simulink model "InductionHeating_bb_4"  (R2026b)
settings: Solver=FixedStepDiscrete  StopTime=0.008
PostLoadFcn:
  | Ts = 1e-6;Ts_fpga=10e-9;   R=3; Capa=300e-9;L=100e-6;Pejo_factor=1;
InitFcn:
  | Ts = 1e-6;Ts_fpga=10e-9;   R=3; Capa=300e-9;L=100e-6;Pejo_factor=1;
undefined symbols (not defined in the file or in its folder): DiscIntNeverNeededParam, ee_sli_rtmsupport, gcbh, isSetWhenUndefinedState, MATESOCwDio
libraries: fl_lib x67, nesl_utility x40, hdlsllib x32, simulink x15, eeGeneralControl x9, ee_lib x3
(part 2 of 7)

== system InductionHeating_bb_4/MATEwDiode ==
  note: mate_diode2.slx for diodes
  g : Inport
  Input : Inport  Port=2
  rl : Inport  Port=3
  C1 : Subsystem  AncestorBlock=simetranss/FPGA/Variable discrete RLC  mask(Discrete variable High Accuracy Series RL or Parallel RC branch){typ=Parallel RC, discmeth=Trapezoidal, Lon=1e-6, R=inf, L=10e-6, Capa=300e-9, sbrl=on, Ts=Ts, showV=off, showI=off}
      mask prompts: typ "Element type"; discmeth "Discretization"; Lon "Switch equivalent ON inductance (H)"; R "Resistor resistance (Ohms)"; L "Inductor inductance (H)"; Capa "Capacitor capacitance (F)"; sbrl "Use signal-based RLC values"; Ts "Sample Time (s)"; showV "Show voltage port"; showI "Show current port"
      mask help:
      | This model implements a discretized  Series RL or Parallel RC branch that is on-line modifiable.
      |
      | On-line modifiable:  RLC parameters can be modified during simulation.
      |
      | Choice of discretization method: Backward Euler (order 1) , Trapzoidal method (order 2) or Radau IIA (5th order)
      |
      | Use with R=0 (Series RL) to obtain a simple inductor.
      | Use with R=inf (Parallel RC) to obtain a simple capacitor.
      |
      | The block can also inplement a Pejovic Switch with the inductance parameter value for ON state. In this case, the resistance is set to 0 internally and capacitance C=Ts*Ts/L and Backward Euler is used.
      mask init:
      | block=gcb;
      | Xcomp=0;
      | s1=0;s2=0;s3=0;s4=0;r1=0;r2=0;l1=0;l2=0;
      | c1=0;c2=0;c3=0;c4=0;x1=0;x2=0;x3=0;x4=0;
      | 
      | MaskEnables =get_param (block ,'MaskEnables' ); 
      | discm=get_param(block,"discmeth");
      | if isequal(get_param(block,"discmeth"),'Backward Euler')
      |     dd=1;
      |     ddi=1;
      | elseif isequal(get_param(block,"discmeth"),'Trapezoidal')
      |     dd=2;
      |     ddi=2;
      | else
      |     dd=5;
      |     ddi=3;
      | end
      | sst=0;
      | br_typ=0;
      | is_sw=0;
      | 
      | % if isequal(get_param(block,"traprule"),'on')
      | %     Trapfactor=2;
      | % else
      | %     Trapfactor=1;
      | % end
      | RootMatch=0;
      | Ihist=0;
      | 
      | if isequal(get_param(block,"showV"),'on')
      |         replace_block (block ,'Followlinks' ,'on' ,'Name' ,'v' ,'BlockType' ,'Terminator' ,'Outport' ,'noprompt' ); 
      | else
      |         replace_block (block ,'Followlinks' ,'on' ,'Name' ,'v' ,'BlockType' ,'Outport' ,'Terminator' ,'noprompt' ); 
      | end
      | if isequal(get_param(block,"showI"),'on')
      |         replace_block (block ,'Followlinks' ,'on' ,'Name' ,'i' ,'BlockType' ,'Terminator' ,'Outport' ,'noprompt' ); 
      | else
      |         replace_block (block ,'Followlinks' ,'on' ,'Name' ,'i' ,'BlockType' ,'Outport' ,'Terminator' ,'noprompt' ); 
      | end
      | 
      | if isequal(get_param(block,"sbrl"),'on')
      |     replace_block (block ,'Followlinks' ,'on' ,'Name' ,'rlc' ,'BlockType' ,'Constant' ,'Inport' ,'noprompt' );
      |     MaskEnables {4 }='off' ;
      |     MaskEnables {5 }='off' ;
      |     MaskEnables {6 }='off' ;
      | else
      |     replace_block (block ,'Followlinks' ,'on' ,'Name' ,'rlc' ,'BlockType' ,'Inport' ,'Constant' ,'noprompt' );
      |     MaskEnables {4 }='on' ;
      |     MaskEnables {5 }='on' ;
      |     MaskEnables {6 }='on' ;
      | end
      | 
      | 
      | 
      | 
      | 
      | 
      | set_param (block ,'MaskEnables' ,MaskEnables ); 
      | qq='x';
      | 
      | typp=get_param(block,'typ');
      | % bp=get_param(block,'pcbp');
      | if isequal(typp,'Pejovic Switch')
      |     replace_block (block ,'Followlinks' ,'on' ,'Name' ,'gate' ,'BlockType' ,'Constant' ,'Inport' ,'noprompt' ); 
      |     %replace_block (block ,'Followlinks' ,'on' ,'Name' ,'init_in' ,'BlockType' ,'Inport' ,'Constant' ,'noprompt'  );
      |     %replace_block (block ,'Followlinks' ,'on' ,'Name' ,'init_out' ,'BlockType' ,'Outport' ,'Terminator' ,'noprompt'  );
      |     Rsw=Lon/Ts;
      |     txt='Switch';
      |     [s1,s2,s3,s4,r1,r2,l1,l2,c1,c2,c3,c4] = MATEdrawRLC('Series RLC Branch',0,1,0,'Open circuit');
      |     c2=[0 -20];
      |     c1=[30 120];
      |     qq='Switch';
      | % MaskEnables {2 }='on' ; 
      | % MaskEnables {3 }='off' ; 
      | % MaskEnables {4 }='off' ; 
      | % MaskEnables {5 }='off' ; 
      | % MaskEnables {6 }='off' ; 
      | % MaskEnables {8 }='off' ;
      | %force Backward Euler
      |     set_param(block,"discmeth",'Backward Euler')
      |     dd=1;
      |     ddi=1;
      |     is_sw=1;
      |     br_typ=0; % use Z=L/h 
      |  
      | elseif isequal(typp,'Inductor')
      |     replace_block (block ,'Followlinks' ,'on' ,'Name' ,'gate' ,'BlockType' ,'Inport' ,'Constant' ,'noprompt' ); 
      |     set_param([block '/gate'],'Value','1');
      |     replace_block (block ,'Followlinks' ,'on' ,'Name' ,'init_in' ,'BlockType' ,'Inport' ,'Constant' ,'noprompt'  ); 
      |     replace_block (block ,'Followlinks' ,'on' ,'Name' ,'init_out' ,'BlockType' ,'Outport' ,'Terminator' ,'noprompt'  );
      |  
      | 
      |     qq='Inductor';
      | % MaskEnables {2 }='off' ; 
      | % MaskEnables {3 }='on' ; 
      | % MaskEnables {4 }='off' ; 
      | % MaskEnables {5 }='on' ; 
      | % MaskEnables {6 }='off' ; 
      | % MaskEnables {8 }='off' ;
      |     x1=0;x2=0;x3=0;x4=0;
      |     if dd==5
      |         warning('Setting Inductor to Trapezoidal discretization');
      |         set_param(block,"discmeth",'Trapezoidal')
      |         dd=2;
      |     end
      |     [s1,s2,s3,s4,r1,r2,l1,l2,c1,c2,c3,c4] = MATEdrawRLC('Series RLC Branch',0,1,0,'L');
      |     [Ad,Bd1,Bd2,Cd,Dd,Y]=discRL(0,1/L,1,0,Ts,dd);
      |     Rsw=1/Y;
      | elseif isequal(typp,'Series RL')
      |     replace_block (block ,'Followlinks' ,'on' ,'Name' ,'gate' ,'BlockType' ,'Inport' ,'Constant' ,'noprompt' ); 
      |     set_param([block '/gate'],'Value','1');
      |     %replace_block (block ,'Followlinks' ,'on' ,'Name' ,'init_in' ,'BlockType' ,'Inport' ,'Constant' ,'noprompt'  ); 
      |     %replace_block (block ,'Followlinks' ,'on' ,'Name' ,'init_out' ,'BlockType' ,'Outport' ,'Terminator' ,'noprompt'  );
      | 
      |     [Ad,Bd1,Bd2,Cd,Dd,Y]=discRL(-R/L,1/L,1,0,Ts,dd);
      |     Rsw=1/Y;
      |     qq='Series RL';
      |     br_typ=0;
      |     sst=0;
      | % MaskEnables {2 }='off' ; 
      | % MaskEnables {3 }='on' ; 
      | % MaskEnables {4 }='off' ; 
      | if isequal(get_param(block,"sbrl"),'off')
      |   MaskEnables {4 }='on' ; 
      |   MaskEnables {5 }='on' ; 
      |   MaskEnables {6 }='off' ; 
      | end
      | % MaskEnables {8 }='off' ;
      |     x1=0;x2=0;x3=0;x4=0;
      |     [s1,s2,s3,s4,r1,r2,l1,l2,c1,c2,c3,c4] = MATEdrawRLC('Series RLC Branch',1,1,0,'RL');
      |     
      |     
      | elseif isequal(typp,'Parallel RC')
      |     replace_block (block ,'Followlinks' ,'on' ,'Name' ,'gate' ,'BlockType' ,'Inport' ,'Constant' ,'noprompt' ); 
      |     set_param([block '/gate'],'Value','0');
      |     %replace_block (block ,'Followlinks' ,'on' ,'Name' ,'init_in' ,'BlockType' ,'Inport' ,'Constant' ,'noprompt'  );
      |     %replace_block (block ,'Followlinks' ,'on' ,'Name' ,'init_out' ,'BlockType' ,'Outport' ,'Terminator' ,'noprompt'  );
      | if R<1e-6
      |     warndlg(['Resistance of RC block: ' block ' is very low for a Parallel RC Branch. Set R=inf if you really want an ideal capacitor with no parallel resistor.'],'MATE warning');
      | end
      |     qq='Capacitor';
      | % MaskEnables {2 }='off' ; 
      | % MaskEnables {3 }='off' ; 
      | % MaskEnables {4 }='on' ; 
      | if isequal(get_param(block,"sbrl"),'off')
      |   MaskEnables {4 }='on' ; 
      |   MaskEnables {5 }='off' ; 
      |   MaskEnables {6 }='on' ; 
      | end
      | 
      | % MaskEnables {8 }='off' ;
      |     % if dd==5 
      |     %     warning('Very low resistance. Setting Capacitor to Trapezoidal discretization');
      |     %     set_param(block,"discmeth",'Trapezoidal')
      |     %     dd=2;
      |     % end
      |     sst=1;
      |     br_typ=1;
      | 
      |     [Ad,Bd1,Bd2,Cd,Dd,Y]=discRL(-1/R/Capa,1/Capa,1,0,Ts,dd);
      |     Rsw=Y;
      | 
      |     if R>1e8
      |             [s1,s2,s3,s4,r1,r2,l1,l2,c1,c2,c3,c4,x1,x2,x3,x4] = MATEdrawRLC('Parallel RLC Branch',0,0,1,'C');
      |                 
      |     else
      |             [s1,s2,s3,s4,r1,r2,l1,l2,c1,c2,c3,c4,x1,x2,x3,x4] = MATEdrawRLC('Parallel RLC Branch',1,0,1,'RC');
      |                  s1=-20;s2=-120;s3=220;s4=120; %reframe
      | 
      |     end
      | 
      | 
      | elseif isequal(typp,'2-level inverter switch')
      |     replace_block (block ,'Followlinks' ,'on' ,'Name' ,'gate' ,'BlockType' ,'Constant' ,'Inport' ,'noprompt' ); 
      |     replace_block (block ,'Followlinks' ,'on' ,'Name' ,'init_in' ,'BlockType' ,'Constant' ,'Inport','noprompt'  );
      |     replace_block (block ,'Followlinks' ,'on' ,'Name' ,'init_out' ,'BlockType' ,'Terminator' ,'Outport' ,'noprompt'  );
      |     Rsw=Lon/Ts;
      |     txt='Inverter half';
      |     Xcomp=1;
      |     qq='Pejo Inverter Half';
      |     %force Backward Euler
      | set_param(block,'traprule','off');
      | % MaskEnables {2 }='on' ; 
      | % MaskEnables {3 }='off' ; 
      | % MaskEnables {4 }='off' ; 
      | % MaskEnables {5 }='off' ; 
      | % MaskEnables {6 }='off' ; 
      | % MaskEnables {8 }='on' ;
      |         [s1,s2,s3,s4,r1,r2,l1,l2,c1,c2,c3,c4] = MATEdrawRLC('Series RLC Branch',0,1,0,'Open circuit');
      |     c2=[0 -20];
      |     c1=[30 120];
      |         if dd==5  ||  dd==2
      |         set_param(block,"discmeth",'Backward Euler')
      |         dd=1;
      |         end
      | 
      | else
      | end
      | 
      | % if isequal(typp,'2-level inverter switch')  && isequal(bp,'on')
      | %         replace_block (block ,'Followlinks' ,'on' ,'Name' ,'Bypass' ,'BlockType' ,'Ground' ,'Inport' ,'noprompt' ); 
      | % else
      | %         replace_block (block ,'Followlinks' ,'on' ,'Name' ,'Bypass' ,'BlockType' ,'Inport' ,'Ground' ,'noprompt' ); 
      | % end
      | 
      | MaskEnables {7 }='on' ; 
      | set_param (block ,'MaskEnables' ,MaskEnables ); 
      | 
      | 
      | if Ts>2e-6
      |     %warndlg(['Sample Time of ' num2str(Ts) ' s. may be somehow large for the Pejovic switch to be accurate. Sample time below 2 us are recommended.'])
      | end
      mask TypeOptions typ: Series RL | Parallel RC | Pejovic Switch
      mask TypeOptions discmeth: Backward Euler | Trapezoidal | Radau IIA 5th order
      mask DialogControl Control2 Prompt: The above RLC parameters will be used as default in SoC
      mask DialogControl Yvalue Prompt: tmp
      mask Display:
      | plot(s1,s2,s3,s4,r1,r2,l1,l2,c1,c2,c3,c4,x1,x2,x3,x4);
      | color('blue')
      | port_label('LConn',1,'+')
      | disp([qq  10 10])
  C2 : Subsystem  AncestorBlock=simetranss/FPGA/Variable discrete RLC  mask(Discrete variable High Accuracy Series RL or Parallel RC branch){typ=Parallel RC, discmeth=Trapezoidal, Lon=1e-6, R=inf, L=100e-6, Capa=300e-9, sbrl=on, Ts=Ts, showV=off, showI=off}
      mask prompts: typ "Element type"; discmeth "Discretization"; Lon "Switch equivalent ON inductance (H)"; R "Resistor resistance (Ohms)"; L "Inductor inductance (H)"; Capa "Capacitor capacitance (F)"; sbrl "Use signal-based RLC values"; Ts "Sample Time (s)"; showV "Show voltage port"; showI "Show current port"
      mask help:
      | This model implements a discretized  Series RL or Parallel RC branch that is on-line modifiable.
      |
      | On-line modifiable:  RLC parameters can be modified during simulation.
      |
      | Choice of discretization method: Backward Euler (order 1) , Trapzoidal method (order 2) or Radau IIA (5th order)
      |
      | Use with R=0 (Series RL) to obtain a simple inductor.
      | Use with R=inf (Parallel RC) to obtain a simple capacitor.
      |
      | The block can also inplement a Pejovic Switch with the inductance parameter value for ON state. In this case, the resistance is set to 0 internally and capacitance C=Ts*Ts/L and Backward Euler is used.
      mask init: same as InductionHeating_bb_4/MATEwDiode/C1
      mask TypeOptions typ: Series RL | Parallel RC | Pejovic Switch
      mask TypeOptions discmeth: Backward Euler | Trapezoidal | Radau IIA 5th order
      mask DialogControl Control2 Prompt: The above RLC parameters will be used as default in SoC
      mask DialogControl Yvalue Prompt: tmp
      mask Display:
      | plot(s1,s2,s3,s4,r1,r2,l1,l2,c1,c2,c3,c4,x1,x2,x3,x4);
      | color('blue')
      | port_label('LConn',1,'+')
      | disp([qq  10 10])
  Cdc : Subsystem  AncestorBlock=simetranss/FPGA/Variable discrete RLC  mask(Discrete variable High Accuracy Series RL or Parallel RC branch){typ=Parallel RC, discmeth=Trapezoidal, Lon=1e-6, R=inf, L=10e-6, Capa=500e-6, sbrl=off, Ts=Ts, showV=off, showI=off}
      mask prompts: typ "Element type"; discmeth "Discretization"; Lon "Switch equivalent ON inductance (H)"; R "Resistor resistance (Ohms)"; L "Inductor inductance (H)"; Capa "Capacitor capacitance (F)"; sbrl "Use signal-based RLC values"; Ts "Sample Time (s)"; showV "Show voltage port"; showI "Show current port"
      mask help:
      | This model implements a discretized  Series RL or Parallel RC branch that is on-line modifiable.
      |
      | On-line modifiable:  RLC parameters can be modified during simulation.
      |
      | Choice of discretization method: Backward Euler (order 1) , Trapzoidal method (order 2) or Radau IIA (5th order)
      |
      | Use with R=0 (Series RL) to obtain a simple inductor.
      | Use with R=inf (Parallel RC) to obtain a simple capacitor.
      |
      | The block can also inplement a Pejovic Switch with the inductance parameter value for ON state. In this case, the resistance is set to 0 internally and capacitance C=Ts*Ts/L and Backward Euler is used.
      mask init: same as InductionHeating_bb_4/MATEwDiode/C1
      mask TypeOptions typ: Series RL | Parallel RC | Pejovic Switch
      mask TypeOptions discmeth: Backward Euler | Trapezoidal | Radau IIA 5th order
      mask DialogControl Control2 Prompt: The above RLC parameters will be used as default in SoC
      mask DialogControl Yvalue Prompt: tmp
      mask Display:
      | plot(s1,s2,s3,s4,r1,r2,l1,l2,c1,c2,c3,c4,x1,x2,x3,x4);
      | color('blue')
      | port_label('LConn',1,'+')
      | disp([qq  10 10])
  Constant : Constant  Value=200
  Controlled Voltage Source : fl_lib/Electrical/Electrical Sources/Controlled Voltage Source
  Current Sensor : fl_lib/Electrical/Electrical Sensors/Current Sensor
  Diode1 : Subsystem  AncestorBlock=simetranss/FPGA/Diode  mask(MATE Diode (Pejovic-based)){VF=0.8, RON=1e-1, LON=1e-6*Pejo_factor, TS=Ts}
      mask prompts: VF "Threshold voltage (V)"; RON "Conduction resistance (Ohms)"; LON "Pejovic Equivalent Inductance during conduction (H)"; TS "Sample time (s)"
      mask help:
      | Implements a diode using a Pejovic switch model.
      |
      | Diode turns ON when Vdiode> Vthreshold and turns OFF when current is 0.
      |
      | The model is based on a Pejovic switch, with equivalent inductance during conduction Lon equal to Lon/Ts=Ts/Coff
      | where Ts is the sample time in second and Coff is the equivalent capacitance when the diode in not conducting.
  Diode2 : Subsystem  AncestorBlock=simetranss/FPGA/Diode  mask(MATE Diode (Pejovic-based)){VF=0.8, RON=1e-1, LON=1e-6*Pejo_factor, TS=Ts}
      mask prompts: VF "Threshold voltage (V)"; RON "Conduction resistance (Ohms)"; LON "Pejovic Equivalent Inductance during conduction (H)"; TS "Sample time (s)"
      mask help:
      | Implements a diode using a Pejovic switch model.
      |
      | Diode turns ON when Vdiode> Vthreshold and turns OFF when current is 0.
      |
      | The model is based on a Pejovic switch, with equivalent inductance during conduction Lon equal to Lon/Ts=Ts/Coff
      | where Ts is the sample time in second and Coff is the equivalent capacitance when the diode in not conducting.
  Diode3 : Subsystem  AncestorBlock=simetranss/FPGA/Diode  mask(MATE Diode (Pejovic-based)){VF=0.8, RON=1e-1, LON=1e-6*Pejo_factor, TS=Ts}
      mask prompts: VF "Threshold voltage (V)"; RON "Conduction resistance (Ohms)"; LON "Pejovic Equivalent Inductance during conduction (H)"; TS "Sample time (s)"
      mask help:
      | Implements a diode using a Pejovic switch model.
      |
      | Diode turns ON when Vdiode> Vthreshold and turns OFF when current is 0.
      |
      | The model is based on a Pejovic switch, with equivalent inductance during conduction Lon equal to Lon/Ts=Ts/Coff
      | where Ts is the sample time in second and Coff is the equivalent capacitance when the diode in not conducting.
  Diode4 : Subsystem  AncestorBlock=simetranss/FPGA/Diode  mask(MATE Diode (Pejovic-based)){VF=0.8, RON=1e-1, LON=1e-6*Pejo_factor, TS=Ts}
      mask prompts: VF "Threshold voltage (V)"; RON "Conduction resistance (Ohms)"; LON "Pejovic Equivalent Inductance during conduction (H)"; TS "Sample time (s)"
      mask help:
      | Implements a diode using a Pejovic switch model.
      |
      | Diode turns ON when Vdiode> Vthreshold and turns OFF when current is 0.
      |
      | The model is based on a Pejovic switch, with equivalent inductance during conduction Lon equal to Lon/Ts=Ts/Coff
      | where Ts is the sample time in second and Coff is the equivalent capacitance when the diode in not conducting.
  Electrical Reference1 : fl_lib/Electrical/Electrical Elements/Electrical Reference
  Electrical Reference2 : fl_lib/Electrical/Electrical Elements/Electrical Reference
  MATE 2-level inverter : Subsystem  AncestorBlock=simetranss/FPGA/MATE 2-level inverter SWFHIZ  mask(MATE Inverter Switching Function (2-level IGBT/Diode) (1-phase)){Ron=1e-3, Vf=0.8, Gpp=100, Gip=1e-6, Ts=Ts, min_charge=5}
      mask prompts: Ron "Switch Ron (Ohms)"; Vf "Switch forward voltage (V)"; Gpp "Snubber resistance (Ohms)"; Gip "Snubber Capacitor (Ohms)"; Ts "Sample time (s)"; min_charge "Minimum rectifying current (A)"
      mask help:
      | This block implements a two-phase, 2-level inverter as a switching function that is capable of High-impedance emulation and oversampling of gate signals by time-step averaging..
      |
      | The block is Time-Step-Averaing capable meaning that the averaging gate ON-time is averaged at each time step.
      | With this approach, dead-times smaller than the sample time are accurately taken into account.
      | Actual resolution of the inverter is only limited by the sampling of the gate values. In HIL applications, if the gate values are sampled at the FPGA clock resolution, the inverter will accurately compute the load voltage with this precision.
      |
      | The inverter can be in high impedance and rectifying states by selecting correctly the RC snubber. Note that the RC snubber is out of circuit during normal (pulsing) model of the inverter.
      | Typically Rsnubber=L_load/Ts , then adjust Csnubber so Rsnubber*Csnubber=2*Ts.
      | On FPGAs, at time step of 1 micro-seconds, R=1kOhms and C=0.1uF are often good.
      |
      | Minimum Rectifying current: In passive mode (no IGBT pulsing), this is the minimum rectifying current that is injected to the DC bus. This parameter is used to avoid unrealistic DC-bus charging when the inverter acts as a diode recfifier, especially with low power factor loads. This option have no impact in active control (gate pulsing) mode.
      |
      | The block has a constant admittance and is suitable for HDL coder.
  PS-Simulink Converter2 : nesl_utility/PS-Simulink Converter  PhysicalDomain=network_engine_domain  SubClassName=ps_output  LeftPortType=input  RightPortType=output  PseudoPeriodic=off  Frequencies=[]  VectorFormat=inherit  Unit=inherit  AffineConversion=off
  PS-Simulink Converter3 : nesl_utility/PS-Simulink Converter  PhysicalDomain=network_engine_domain  SubClassName=ps_output  LeftPortType=input  RightPortType=output  PseudoPeriodic=off  Frequencies=[]  VectorFormat=inherit  Unit=inherit  AffineConversion=off
  RC : Constant  Value=[inf 300e-9]  SampleTime=Ts
  RC1 : Constant  Value=[inf 500e-6]  SampleTime=Ts
  RL1 : Subsystem  AncestorBlock=simetranss/FPGA/Variable discrete RLC  mask(Discrete variable High Accuracy Series RL or Parallel RC branch){typ=Series RL, discmeth=Trapezoidal, Lon=1e-6, R=3, L=100e-6, Capa=300e-6, sbrl=on, Ts=Ts, showV=off, showI=off, fpga_varY=on}
      mask prompts: typ "Element type"; discmeth "Discretization"; Lon "Switch equivalent ON inductance (H)"; R "Resistor resistance (Ohms)"; L "Inductor inductance (H)"; Capa "Capacitor capacitance (F)"; sbrl "Use signal-based RLC values"; Ts "Sample Time (s)"; showV "Show voltage port"; showI "Show current port"; fpga_varY "FPGA on-line variable value element (only 1 per circuit)"
      mask help:
      | This model implements a discretized  Series RL or Parallel RC branch that is on-line modifiable.
      |
      | On-line modifiable:  RLC parameters can be modified during simulation.
      |
      | Choice of discretization method: Backward Euler (order 1) , Trapzoidal method (order 2) or Radau IIA (5th order)
      |
      | Use with R=0 (Series RL) to obtain a simple inductor.
      | Use with R=inf (Parallel RC) to obtain a simple capacitor.
      |
      | The block can also inplement a Pejovic Switch with the inductance parameter value for ON state. In this case, the resistance is set to 0 internally and capacitance C=Ts*Ts/L and Backward Euler is used.
      |
      | FPGA on-line variable value element (only 1 per circuit): this check identify the element as on-line variable in the FPGA simulation. On FPGA, there can be only 1 of these (in the 2026 implementation). This flag will indicate to the solver that the corresponding internal discrete resistance is to be disregarded for the initial D circuit matrix and to be included during execution afterward.
      mask init: same as InductionHeating_bb_4/MATEwDiode/C1
      mask TypeOptions typ: Series RL | Parallel RC | Pejovic Switch
      mask TypeOptions discmeth: Backward Euler | Trapezoidal | Radau IIA 5th order
      mask DialogControl Control2 Prompt: The above RLC parameters will be used as default in SoC
      mask DialogControl Yvalue Prompt: tmp
      mask Display:
      | plot(s1,s2,s3,s4,r1,r2,l1,l2,c1,c2,c3,c4,x1,x2,x3,x4);
      | color('blue')
      | port_label('LConn',1,'+')
      | disp([qq  10 10])
  R_Conv_in3 : fl_lib/Electrical/Electrical Elements/Resistor  R=0.01 Ohm  i_specify=off  i_priority=None  i=0 A  i_nominal_specify=off  i_nominal_value=1  i_nominal_unit=A  v_specify=off  v_priority=None  v=0 V  v_nominal_specify=off  v_nominal_value=1  v_nominal_unit=V
      settings: AttributesFormatString=%<R> %<R_unit>
  R_Line_in2 : fl_lib/Electrical/Electrical Elements/Resistor  R=0.01 Ohm  i_specify=off  i_priority=None  i=0 A  i_nominal_specify=off  i_nominal_value=1  i_nominal_unit=A  v_specify=off  v_priority=None  v=0 V  v_nominal_specify=off  v_nominal_value=1  v_nominal_unit=V
      settings: AttributesFormatString=%<R> %<R_unit>
  Resistor1 : fl_lib/Electrical/Electrical Elements/Resistor  R=1e7 Ohm  i_specify=off  i_priority=None  i=0 A  i_nominal_specify=off  i_nominal_value=1  i_nominal_unit=A  v_specify=off  v_priority=None  v=0 V  v_nominal_specify=off  v_nominal_value=1  v_nominal_unit=V
  Resistor2 : fl_lib/Electrical/Electrical Elements/Resistor  R=1000000 Ohm  i_specify=off  i_priority=None  i=0 A  i_nominal_specify=off  i_nominal_value=1  i_nominal_unit=A  v_specify=off  v_priority=None  v=0 V  v_nominal_specify=off  v_nominal_value=1  v_nominal_unit=V
  Simulink-PS Converter1 : nesl_utility/Simulink-PS Converter  PhysicalDomain=network_engine_domain  SubClassName=ps_input  LeftPortType=input  RightPortType=output  PseudoPeriodic=off  Frequencies=[]  NoiseDistribution=none  NoiseParameters=[]  Unit=1  AffineConversion=off  FilteringAndDerivatives=provide  SimscapeFilterOrder=1  InputFilterTimeConstant=0.001  UdotUserProvided=0
  Simulink-PS Converter2 : nesl_utility/Simulink-PS Converter  PhysicalDomain=network_engine_domain  SubClassName=ps_input  LeftPortType=input  RightPortType=output  PseudoPeriodic=off  Frequencies=[]  NoiseDistribution=none  NoiseParameters=[]  Unit=1  AffineConversion=off  FilteringAndDerivatives=provide  SimscapeFilterOrder=1  InputFilterTimeConstant=0.001  UdotUserProvided=0
  Solver Configuration1 : nesl_utility/Solver Configuration  PhysicalDomain=network_engine_domain  SubClassName=solver  LeftPortType=input  RightPortType=generic  Tones=[]  Harmonics=[]  SimulateNoise=off  Profile=off  UseLocalSampling=off  EnableSwitchedLinearOptims=on  FrequencyDomain=off  UseCCode=off  RelTol=0.001  AbsTol=1e-06  MinStep=1e-09  ToWorkspace=off  RevertToSquareIcSolve=off  NumHomotopyIterations=100  PhasorMode=off  PhasorModeNumHarmonics=1  ConsistencySolver=NEWTON_FTOL  CanonicalOrdering=UNORDERED  OptimizeIntermediates=UNOPTIMIZED  MulticoreSolverChoice=BACKWARD_EULER  IndexReductionMethod=DerivativeReplacement  DoDC=off  ResidualTolerance=1e-09  ConsistencyTolSource=GLOBAL  ConsistencyAbsTol=0.001  ConsistencyRelTol=0.001  ConsistencyTolFactor=0.001  UseLocalSolver=on  LocalSolverChoice=NE_BACKWARD_EULER_ADVANCER  ResolveIndetEquations=on  FunctionEvalNumThread=1  LocalSolverSampleTime=1e-6  DoFixedCost=on  MaxNonlinIter=1  MaxModeIter=2  ComputeImpulses=off  ImpulseIterations=2  LinearAlgebra=auto  LinearAlgebraNumThread=0  EquationFormulation=NE_TIME_EF  DelaysMemoryBudget=1024  AutomaticFiltering=on  FilteringTimeConstant=0.001  PartitionStorageMethod=AS_NEEDED  PartitionMemoryBudget=1024  PartitionMethod=BALANCED  MultibodyUseLocalSolver=off  MultibodyLocalSolverChoice=ODE1  MultibodyLocalSolverSampleTime=0.001
  Subsystem3 : Subsystem
      settings: PortSchema="{\"entries\":[{\"content\":{\"sides\":[{\"content\":{\"connectorIds\":[\"LConn1\"]},\"type\":\"ConnectorPlacement.EquallySpacedRectSide\",\"uuid\":\"076679af-cf2d-42cc-92f3-c0233f61b32a\"},{\"content\":{\"connectorIds\":[\"RConn1\"],\"side\":\"RIGHT\"},\"type\":\"ConnectorPlacement.EquallySpacedRectSide\",\"uuid\":\"b256d27d-4c49-40e6-9ef5-c4a9651a2296\"},{\"content\":{\"connectorIds\":[\"Out1\"],\"side\":\"TOP\"},\"type\":\"ConnectorPlacement.EquallySpacedRectSide\",\"uuid\":\"7c2293c3-6569-452f-b68e-58f8d8f046a0\"}]},\"type\":\"ConnectorPlacement.EquallySpacedConnector\",\"uuid\":\"813ba93f-15bf-4e08-b2ea-5f69cefe7eb7\"}],\"packageUris\":[\"http://schema.mathworks.com/mf0/Connector/R2020b\"],\"version\":\"1.0\"}"
  Voltage Sensor1 : fl_lib/Electrical/Electrical Sensors/Voltage Sensor
  iload : Outport
  i_src : Outport  Port=2
  vdc : Outport  Port=3
  wires:
  RC/1 -> C2/1(rlc), C1/1(rlc)
  Subsystem3/1(i) -> iload/1  "iload"
  g/1 -> MATE 2-level inverter/1(g)
  PS-Simulink Converter2/1 -> vdc/1
  Input/1 -> Simulink-PS Converter2/1
  PS-Simulink Converter3/1 -> i_src/1
  RC1/1 -> ?
  rl/1 -> RL1/1(rlc)
  Constant/1 -> Simulink-PS Converter1/1
  connections:
  Voltage Sensor1/RConn2 -- Diode4/LConn1 -- Diode3/LConn1 -- Cdc/RConn1 -- C2/RConn1 -- MATE 2-level inverter/LConn2
  Electrical Reference1/LConn1 -- Resistor1/RConn1
  R_Conv_in3/RConn1 -- C1/LConn1 -- MATE 2-level inverter/LConn1
  Resistor1/LConn1 -- C1/RConn1 -- RL1/RConn1 -- C2/LConn1
  Diode2/RConn1 -- R_Conv_in3/LConn1 -- Voltage Sensor1/LConn1 -- Cdc/LConn1 -- Diode1/RConn1
  Solver Configuration1/RConn1 -- Controlled Voltage Source/RConn2 -- Resistor2/LConn1 -- Diode4/RConn1 -- Diode1/LConn1
  Diode2/LConn1 -- Diode3/RConn1 -- Current Sensor/RConn2
  Voltage Sensor1/RConn1 -- PS-Simulink Converter2/LConn1
  Controlled Voltage Source/LConn1 -- R_Line_in2/LConn1
  Simulink-PS Converter2/RConn1 -- Controlled Voltage Source/RConn1
  Electrical Reference2/LConn1 -- Resistor2/RConn1
  PS-Simulink Converter3/LConn1 -- Current Sensor/RConn1
  R_Line_in2/RConn1 -- Current Sensor/LConn1
  Subsystem3/LConn1 -- MATE 2-level inverter/RConn1
  RL1/LConn1 -- Subsystem3/RConn1

== system InductionHeating_bb_4/PWM_Generator3 ==
  note: be careful with gain in int32: 0.25 transform to 0!!!
  PWMsteps : Inport
  PWMstepsON : Inport  Port=2
  deatime(s) : Inport  Port=3
  enable : Inport  Port=4
  Data Type Conversion1 : DataTypeConversion  OutDataTypeStr=single  RndMeth=Nearest  SaturateOnIntegerOverflow=off
  Discrete Triangular-Waveform Generator : Subsystem
  Discrete-Time Integrator : DiscreteIntegrator  gainval=1  ExternalReset=level  SampleTime=Ts  LimitOutput=on  ICPrevOutput=DiscIntNeverNeededParam  ICPrevScaledInput=DiscIntNeverNeededParam
  Divide1 : Product
  Logical Operator1 : Logic  Operator=NOT  AllPortsSameDT=off  OutDataTypeStr=boolean
  Logical Operator2 : Logic  AllPortsSameDT=off  OutDataTypeStr=boolean
  Logical Operator3 : Logic  Operator=NOT  AllPortsSameDT=off  OutDataTypeStr=boolean
  Mux1 : Mux  Inputs=2
  Relational Operator1 : RelationalOperator  Operator=>  OutDataTypeStr=boolean  RndMeth=Simplest  InputSameDT=off
  gate : Outport  VectorParamsAs1DForOutWhenUnconnected=off
  wires:
  Logical Operator2/1 -> Divide1/2
  Divide1/1 -> gate/1
  enable/1 -> Divide1/1
  PWMstepsON/1 -> Discrete Triangular-Waveform Generator/2(stepON)
  PWMsteps/1 -> Discrete Triangular-Waveform Generator/1(steps)
  ? -> ?
  Discrete Triangular-Waveform Generator/1(pulse) -> Mux1/1, Logical Operator1/1
  Discrete-Time Integrator/1 -> Relational Operator1/1
  Relational Operator1/1 -> Logical Operator2/1
  Logical Operator3/1 -> Discrete-Time Integrator/2
  Logical Operator1/1 -> Mux1/2
  Mux1/1 -> Data Type Conversion1/1, Logical Operator3/1, Logical Operator2/2
  Data Type Conversion1/1 -> Discrete-Time Integrator/1  "Simulink-PS Converter1"
  deatime(s)/1 -> Relational Operator1/2

== system InductionHeating_bb_4/Subsystem ==
  In1 : Inport
  2 : Constant  SampleTime=Ts
  Divide1 : Product  Inputs=*/
  Gain4 : Gain  Gain=Ts
  Out1 : Outport
  wires:
  In1/1 -> Gain4/1
  Gain4/1 -> Divide1/2
  2/1 -> Divide1/1
  Divide1/1 -> Out1/1
